simulink model "FOC_Core_OL"  (R2025b)
settings: Solver=FixedStepDiscrete  StartTime=0.0  StopTime=Tstop  FixedStep=8e-05  RelTol=1e-3
undefined symbols (not defined in the file): p
settings Model: Creator=dehc5899  LastModifiedBy=dehc5899
settings SolverCC: AutoInsertRateTranBlk=on
settings DataIOCC: SaveOutput=off  SaveTime=off
settings OptimizationCC: DefaultParameterBehavior=Inlined  EnhancedBackFolding=on  PassReuseOutputArgsAs=Individual arguments  ZeroExternalMemoryAtStartup=off  ZeroInternalMemoryAtStartup=off  OptimizeBlockOrder=speed  DifferentSizesBufferReuse=on  OptimizationCustomize=off  EfficientTunableParamExpr=on
settings DebuggingCC: UnderspecifiedInitializationDetection=Classic  ParameterTunabilityLossMsg=error  BusObjectLabelMismatch=none
settings HardwareCC: ProdBitPerPointer=32.0  ProdBitPerSizeT=32.0  ProdBitPerPtrDiffT=32.0  ProdLargestAtomicInteger=Long  ProdLargestAtomicFloat=Double  ProdWordSize=32.0  ProdHWDeviceType=ARM Compatible->ARM Cortex-M
settings SFSimCC: MATLABDynamicMemAlloc=off
settings RTWCC: SystemTargetFile=ert.tlc  GenCodeOnly=on  GenerateMakefile=off  TemplateMakefile=RTW.MSVCBuild  GenerateReport=on  Description=Create Visual C/C++ Solution File for Embedded Coder
settings CodeAppCC: ForceParamTrailComments=on  IgnoreCustomStorageClasses=off  OperatorAnnotations=on  SimulinkDataObjDesc=on  SFDataObjDesc=on  InsertBlockDesc=on
settings ERTTargetCC: ERTCustomFileTemplate=example_file_process.tlc  TargetLangStandard=C99 (ISO)  GenerateSampleERTMain=on  SupportAbsoluteTime=off  SupportNonFinite=off  SupportComplex=off

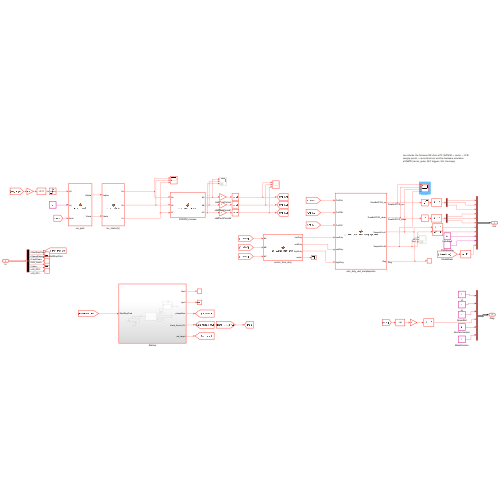
[thumbnail: Simulink's stored preview of the top-level diagram]
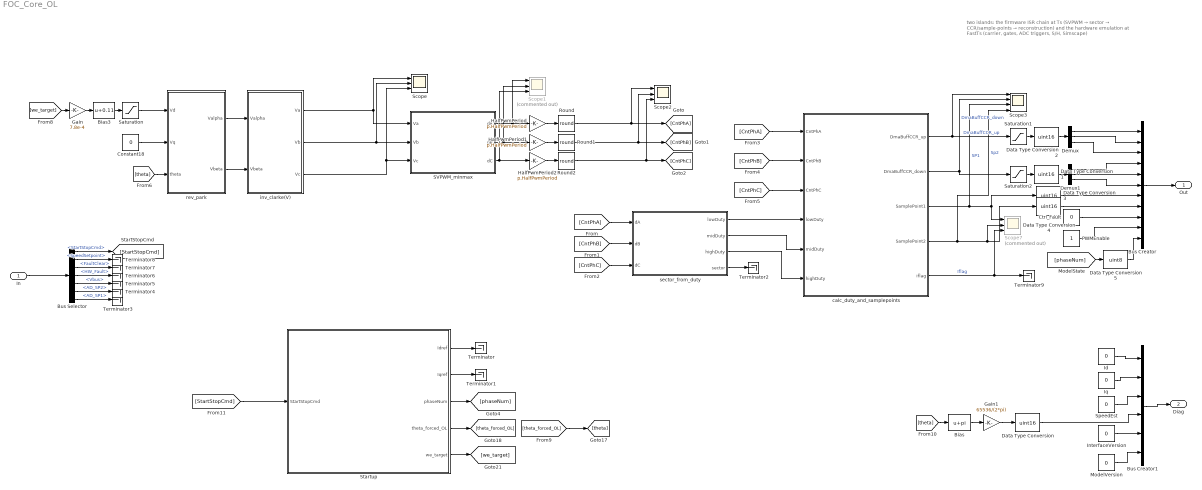
== system FOC_Core_OL ==
  note: two islands: the firmware ISR chain at Ts (SVPWM → sector → CCR/sample-points → reconstruction) and the hardware emulation at FastTs (carrier, gates, ADC triggers, S/H, Simscape)
  In : Inport  OutDataTypeStr=Bus: FOC_Inputs_t
  Bias : Bias  Bias=pi  SaturateOnIntegerOverflow=off
  Bias3 : Bias  Bias=0.11  SaturateOnIntegerOverflow=off
  Bus Creator : BusCreator  Inputs=11  OutDataTypeStr=Bus: FOC_Outputs_t
  Bus Creator1 : BusCreator  Inputs=6  OutDataTypeStr=Bus: FOC_ModelDiag_t
  Bus Selector : BusSelector  OutputSignals=StartStopCmd,SpeedSetpoint,FaultClear,HW_Fault,Vbus,AD_SP2,AD_SP1
  Constant18 : Constant  Value=0
  Ctrl_Fault : Constant  Value=0  OutDataTypeStr=uint16
  Data Type Conversion : DataTypeConversion  OutDataTypeStr=uint16  RndMeth=Floor
  Data Type Conversion{1..4} (4 alike) : DataTypeConversion  OutDataTypeStr=uint16  RndMeth=Nearest
  Data Type Conversion5 : DataTypeConversion  OutDataTypeStr=uint8  RndMeth=Nearest
  Demux : Demux  Outputs=3
  Demux1 : Demux  Outputs=3
  Gain : Gain  Gain=7.8e-4
  Gain1 : Gain  Gain=65536/(2*pi)
  HalfPwmPeriod : Gain  Gain=p.HalfPwmPeriod
  HalfPwmPeriod1 : Gain  Gain=p.HalfPwmPeriod
  HalfPwmPeriod2 : Gain  Gain=p.HalfPwmPeriod
  Id : Constant  Value=0  OutDataTypeStr=int16
  InterfaceVersion : Constant  Value=0  OutDataTypeStr=uint16
  Iq : Constant  Value=0  OutDataTypeStr=int16
  ModelVersion : Constant  Value=0  OutDataTypeStr=uint16
  PWMEnable : Constant  OutDataTypeStr=uint8
  Round : Rounding  Operator=round
  Round1 : Rounding  Operator=round
  Round2 : Rounding  Operator=round
  SVPWM_minmax : MATLAB Function  TreatAsAtomicUnit=on
  Saturation : Saturate  UpperLimit=0.9  LowerLimit=0
  Saturation1 : Saturate  UpperLimit=5120  LowerLimit=0
  Saturation2 : Saturate  UpperLimit=5120  LowerLimit=0
  Scope : Scope  NumInputPorts=3
      settings: ActiveDisplayYMinimum=-1.7670802058532755  ActiveDisplayYMaximum=1.7615871298568744  DataLoggingVariableName=ScopeData24
  Scope1 : Scope  Commented=on  NumInputPorts=3
      settings: ActiveDisplayYMinimum=0.36044361461932012  ActiveDisplayYMaximum=0.40645121419536845  DataLoggingVariableName=ScopeData26
  Scope2 : Scope  NumInputPorts=3
      settings: ActiveDisplayYMinimum=1487.5  ActiveDisplayYMaximum=5312.5  DataLoggingVariableName=ScopeData27
  Scope3 : Scope  NumInputPorts=4
      settings: ActiveDisplayYMinimum=1272.0361133462177  ActiveDisplayYMaximum=3996.5603864724189  DataLoggingVariableName=ScopeData29
  Scope7 : Scope  Commented=on  NumInputPorts=3
      settings: ActiveDisplayYMinimum=669.00000000000011  ActiveDisplayYMaximum=6049  DataLoggingVariableName=ScopeData30
  SpeedEst : Constant  Value=0  OutDataTypeStr=int16
  Startup : Subsystem
  Terminator{,1..9} (10 alike) : Terminator
  calc_duty_and_samplepoints : MATLAB Function  TreatAsAtomicUnit=on
  inv_clarke(V) : MATLAB Function  TreatAsAtomicUnit=on
  rev_park : MATLAB Function  TreatAsAtomicUnit=on
  sector_from_duty : MATLAB Function  TreatAsAtomicUnit=on
  Out : Outport  OutDataTypeStr=Bus: FOC_Outputs_t
  Diag : Outport  Port=2  OutDataTypeStr=Bus: FOC_ModelDiag_t
  wires:
  calc_duty_and_samplepoints/3(SamplePoint1) -> Scope3/3, Data Type Conversion3/1, Scope7/1  "SP1"
  SVPWM_minmax/2(dB) -> Scope1/2, HalfPwmPeriod1/1
  HalfPwmPeriod/1 -> Round/1
  sector_from_duty/3(highDuty) -> calc_duty_and_samplepoints/6(highDuty)
  calc_duty_and_samplepoints/4(SamplePoint2) -> Scope3/4, Data Type Conversion4/1, Scope7/2  "Sp2"
  inv_clarke(V)/2(Vb) -> SVPWM_minmax/2(Vb), Scope/2
  [CntPhC] -> sector_from_duty/3(dC)
  inv_clarke(V)/1(Va) -> Scope/1, SVPWM_minmax/1(Va)
  sector_from_duty/4(sector) -> Terminator2/1
  Round/1 -> [CntPhA], Scope2/1
  HalfPwmPeriod2/1 -> Round2/1
  SVPWM_minmax/3(dC) -> Scope1/3, HalfPwmPeriod2/1
  calc_duty_and_samplepoints/2(DmaBuffCCR_down) -> Saturation2/1, Scope3/2  "DmaBuffCCR_down"
  [CntPhB] -> sector_from_duty/2(dB)
  [CntPhB] -> calc_duty_and_samplepoints/2(CntPhB)
  SVPWM_minmax/1(dA) -> Scope1/1, HalfPwmPeriod/1
  calc_duty_and_samplepoints/1(DmaBuffCCR_up) -> Saturation1/1, Scope3/1  "DmaBuffCCR_up"
  [CntPhA] -> sector_from_duty/1(dA)
  inv_clarke(V)/3(Vc) -> SVPWM_minmax/3(Vc), Scope/3
  Round1/1 -> Scope2/2, [CntPhB]
  sector_from_duty/1(lowDuty) -> calc_duty_and_samplepoints/4(lowDuty)
  [CntPhC] -> calc_duty_and_samplepoints/3(CntPhC)
  sector_from_duty/2(midDuty) -> calc_duty_and_samplepoints/5(midDuty)
  [CntPhA] -> calc_duty_and_samplepoints/1(CntPhA)
  HalfPwmPeriod1/1 -> Round1/1
  Round2/1 -> Scope2/3, [CntPhC]
  calc_duty_and_samplepoints/5(iflag) -> Terminator9/1, Scope7/3  "Iflag"
  [we_target] -> Gain/1
  Startup/3(phaseNum) -> [phaseNum]
  Constant18/1 -> rev_park/2(Vq)
  Startup/5(we_target) -> [we_target]
  Gain/1 -> Bias3/1
  [theta_forced_OL] -> [theta]
  Saturation/1 -> rev_park/1(Vd)
  rev_park/1(Valpha) -> inv_clarke(V)/1(Valpha)
  Startup/4(theta_forced_OL) -> [theta_forced_OL]
  rev_park/2(Vbeta) -> inv_clarke(V)/2(Vbeta)
  Startup/2(Iqref) -> Terminator1/1
  [theta] -> rev_park/3(theta)
  Startup/1(Idref) -> Terminator/1
  Bias3/1 -> Saturation/1
  In/1 -> Bus Selector/1
  Bus Selector/7 -> Terminator3/1  "<AD_SP1>"
  Bus Selector/6 -> Terminator4/1  "<AD_SP2>"
  Bus Selector/5 -> Terminator5/1  "<Vbus>"
  Bus Selector/4 -> Terminator6/1  "<HW_Fault>"
  Bus Selector/3 -> Terminator7/1  "<FaultClear>"
  Bus Selector/2 -> Terminator8/1  "<SpeedSetpoint>"
  Bus Selector/1 -> [StartStopCmd]  "<StartStopCmd>"
  Demux/1 -> Bus Creator/1
  Demux/2 -> Bus Creator/2
  Demux/3 -> Bus Creator/3
  Demux1/1 -> Bus Creator/4
  Demux1/2 -> Bus Creator/5
  Demux1/3 -> Bus Creator/6
  Ctrl_Fault/1 -> Bus Creator/9
  PWMEnable/1 -> Bus Creator/10
  [phaseNum] -> Data Type Conversion5/1
  Bus Creator/1 -> Out/1
  Saturation1/1 -> Data Type Conversion2/1
  Saturation2/1 -> Data Type Conversion1/1
  Id/1 -> Bus Creator1/1
  Iq/1 -> Bus Creator1/2
  Bus Creator1/1 -> Diag/1
  InterfaceVersion/1 -> Bus Creator1/5
  ModelVersion/1 -> Bus Creator1/6
  [theta] -> Bias/1
  Bias/1 -> Gain1/1
  Gain1/1 -> Data Type Conversion/1
  Data Type Conversion/1 -> Bus Creator1/4
  [StartStopCmd] -> Startup/1(StartStopCmd)
  SpeedEst/1 -> Bus Creator1/3
  Data Type Conversion1/1 -> Demux1/1
  Data Type Conversion2/1 -> Demux/1
  Data Type Conversion3/1 -> Bus Creator/7
  Data Type Conversion4/1 -> Bus Creator/8
  Data Type Conversion5/1 -> Bus Creator/11

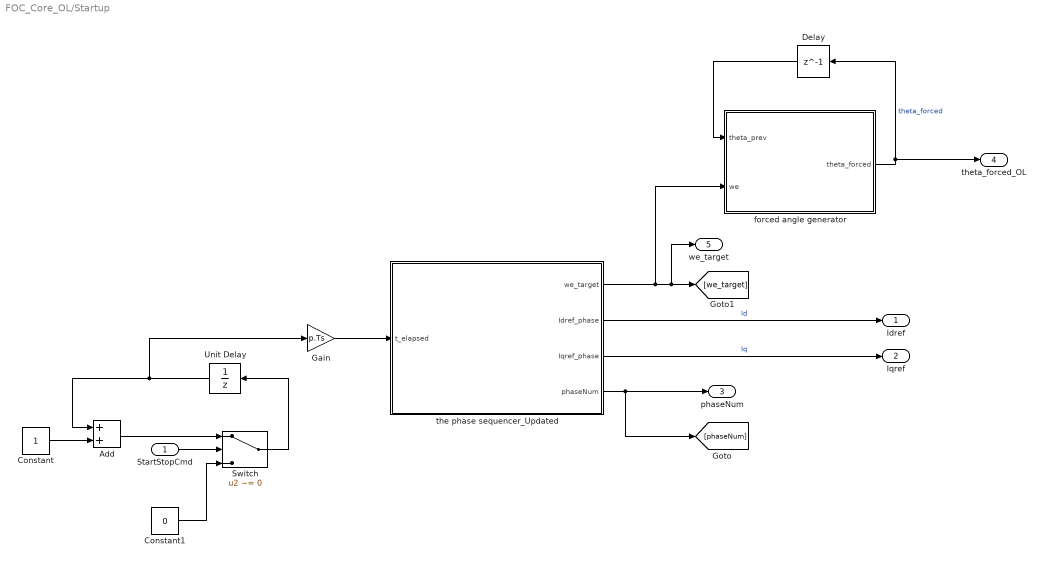
== system FOC_Core_OL/Startup ==
  StartStopCmd : Inport
  Add : Sum
  Constant : Constant  OutDataTypeStr=uint32
  Constant1 : Constant  Value=0  OutDataTypeStr=uint32
  Delay : Delay  DelayLength=1  SampleTime=p.Ts
  Gain : Gain  Gain=p.Ts  ParamDataTypeStr=double  OutDataTypeStr=double
  Switch : Switch  Criteria=u2 ~= 0  SaturateOnIntegerOverflow=off  InputSameDT=off
  Unit Delay : UnitDelay  SampleTime=-1  HasFrameUpgradeWarning=on
  forced angle generator : MATLAB Function  TreatAsAtomicUnit=on
  the phase sequencer_Updated : MATLAB Function  TreatAsAtomicUnit=on
  Idref : Outport
  Iqref : Outport  Port=2
  phaseNum : Outport  Port=3  OutDataTypeStr=double
  theta_forced_OL : Outport  Port=4
  we_target : Outport  Port=5
  wires:
  the phase sequencer_Updated/1(we_target) -> [we_target], we_target/1, forced angle generator/2(we)
  the phase sequencer_Updated/2(Idref_phase) -> Idref/1  "Id"
  the phase sequencer_Updated/3(Iqref_phase) -> Iqref/1  "Iq"
  Delay/1 -> forced angle generator/1(theta_prev)
  forced angle generator/1(theta_forced) -> theta_forced_OL/1, Delay/1  "theta_forced"
  the phase sequencer_Updated/4(phaseNum) -> [phaseNum], phaseNum/1
  Constant/1 -> Add/2
  Unit Delay/1 -> Add/1, Gain/1
  Gain/1 -> the phase sequencer_Updated/1(t_elapsed)
  Add/1 -> Switch/1
  StartStopCmd/1 -> Switch/2
  Constant1/1 -> Switch/3
  Switch/1 -> Unit Delay/1

== matlab function FOC_Core_OL/SVPWM_minmax ==
  data: Va input; dA output; Vb input; Vc input; dB output; dC output
function [dA, dB, dC] = ss_svpwm_minmax(Va, Vb, Vc)
%SS_SVPWM_MINMAX Carrier-based SVPWM via min-max common-mode injection.
%
% Standard trick to get space-vector-equivalent modulation without ever
% computing a vector angle or sector: subtract the average of the largest
% and smallest of the three instantaneous reference voltages from all
% three. That "third-harmonic-like" zero-sequence term cancels line-to-
% line (so it doesn't affect the actual motor voltages) but centers the
% three duty cycles inside the 0..1 carrier range, extending the linear
% modulation range from m=1 (plain sine-triangle) to m=2/sqrt(3)~=1.1547
% (six-step limit) - the same range single-shunt SVPWM assumes.
%
% This is the same formula used inline in
% test_single_shunt_reconstruction.m (and export_for_simulink.m); pulled
% out here so it can be dropped into a Simulink MATLAB Function block and
% reused instead of duplicated.
%
% Va, Vb, Vc : per-unit reference phase voltages, nominally in [-1, 1]
%              (e.g. Va = m*cos(theta_e), 120 deg apart), where m is the
%              modulation index.
%
% dA, dB, dC : duty cycle in [0, 1], ready for the next stage (converting
%              to timer counter/CCR values, i.e. CntPhX = round(dX *
%              Half_PWMPeriod) - NOT done here on purpose, kept as a
%              separate step).

v0 = -(max([Va, Vb, Vc]) + min([Va, Vb, Vc])) / 2;

dA = 0.5 + 0.5 * (Va + v0);
dB = 0.5 + 0.5 * (Vb + v0);
dC = 0.5 + 0.5 * (Vc + v0);

end

== matlab function FOC_Core_OL/calc_duty_and_samplepoints ==
  data: CntPhA input; DmaBuffCCR_up output size=[1 3]; CntPhB input; CntPhC input; lowDuty input; midDuty input; highDuty input; DmaBuffCCR_down output size=[1 3]; SamplePoint1 output; SamplePoint2 output; iflag output; p parameter
function [DmaBuffCCR_up, DmaBuffCCR_down, SamplePoint1, SamplePoint2, iflag] = ...
    ss_calc_duty_and_samplepoints(CntPhA, CntPhB, CntPhC, lowDuty, midDuty, highDuty, p)
%SS_CALC_DUTY_AND_SAMPLEPOINTS MATLAB port of R1_CalcDutyCycles()
% (Src/r1_ps_pwm_curr_fdbk.c, ~lines 1097-1282).
%
% Every PWM period, single-shunt sensing needs two ADC injected
% conversions of the DC-link shunt current, timed to fall inside the two
% "two-phases-on" sub-intervals either side of the mid-duty phase's
% switching edges. Those windows only exist, and are only wide enough to
% trigger + finish a conversion (>= p.TMin ticks), when the three duty
% cycles are far enough apart. Close to a sector boundary (two duties
% nearly equal) the natural window collapses, so this function:
%
%   1) checks the two natural gaps (high-mid, mid-low) against TMin;
%   2) if a gap is too small but can still be opened by shifting the
%      shorter leg's compare value by a few ticks, does so via aShiftval
%      (kept symmetric: +shift in the first half of the center-aligned
%      PWM period, -shift in the second half, so the AVERAGE duty over
%      the full period - and thus the commanded voltage - is unchanged);
%   3) if even that isn't possible (duty pinned near 0% or 100%), marks
%      that phase as unavailable this period (iflag bit cleared) and
%      falls back to one fixed sampling point at mid-period;
%   4) returns iflag (IA_OK/IB_OK/IC_OK bits) telling
%      ss_get_phase_currents() which phase current(s) can be trusted from
%      this period's two ADC samples, and which must fall back to an
%      estimate instead.
%
% Inputs are all timer ticks (see ss_params, matches p.HalfPwmPeriod).
% CntPhA/B/C : commanded compare values (0..p.HalfPwmPeriod)
% lowDuty/midDuty/highDuty : 0-based phase index (0=A,1=B,2=C), from
%                            ss_sector_from_duty
%
% Outputs:
% DmaBuffCCR_up/down : shifted CCR values for the up-count / down-count
%                      half of the period (mirrors DmaBuffCCR[0:2] and
%                      DmaBuffCCR[4:6])
% SamplePoint1/2     : ADC trigger points in timer ticks (TIM1_CH5/CH6)
% iflag              : uint8 bitmask, bit0=IA_OK bit1=IB_OK bit2=IC_OK

IA_OK = uint8(1); IB_OK = uint8(2); IC_OK = uint8(4);
ALFLAG = [IA_OK IB_OK IC_OK];

aCCRval = [CntPhA, CntPhB, CntPhC];
maxVal = highDuty + 1;   % to 1-based MATLAB index
midIdx = midDuty  + 1;
minVal = lowDuty  + 1;

iflag = uint8(0);
aShiftval = [0 0 0];

submax_mid          = aCCRval(maxVal) - aCCRval(midIdx);
submax_mid_deltmin   = submax_mid - p.TMin;
submid_min           = aCCRval(midIdx) - aCCRval(minVal);
submid_min_deltmin   = submid_min - p.TMin;
max_bad_flag = false;
min_bad_flag = false;

if submax_mid_deltmin > 0
    iflag = bitor(iflag, ALFLAG(maxVal));
else
    if (1 - submax_mid_deltmin + aCCRval(maxVal) + p.hTADConv) > p.HalfPwmPeriod
        max_bad_flag = true;            % no room to open a window even after shifting
    else
        iflag = bitor(iflag, ALFLAG(maxVal));
        aShiftval(maxVal) = 1 - submax_mid_deltmin;
    end
end

if submid_min_deltmin > 0
    iflag = bitor(iflag, ALFLAG(minVal));
else
    if (submid_min_deltmin - 1 + aCCRval(minVal)) < 0
        min_bad_flag = true;
    else
        iflag = bitor(iflag, ALFLAG(minVal));
        aShiftval(minVal) = submid_min_deltmin - 1;
    end
end

if (~max_bad_flag) && (~min_bad_flag)
    SamplePoint1 = aCCRval(midIdx) - p.TSample;
    SamplePoint2 = aCCRval(midIdx) + p.TMin - p.TSample;
elseif max_bad_flag && min_bad_flag
    SamplePoint1 = p.HalfPwmPeriod / 2;
    SamplePoint2 = SamplePoint1 + p.TSample + p.hTADConv;
elseif max_bad_flag
    SamplePoint1 = aCCRval(midIdx) - p.TSample;
    SamplePoint2 = aCCRval(midIdx) + p.hTADConv;
else
    SamplePoint2 = aCCRval(midIdx) + p.TMin - p.TSample;
    SamplePoint1 = aCCRval(midIdx);
end


if (SamplePoint2 - SamplePoint1) < p.hTADConv
    iflag = bitand(iflag, ALFLAG(maxVal));
    iflag = bitand(iflag, bitcmp(ALFLAG(minVal)));
    SamplePoint1 = p.HalfPwmPeriod / 2;
    SamplePoint2 = SamplePoint1 + p.TSample + p.hTADConv;
end

if (SamplePoint2 >= p.HalfPwmPeriod) || (SamplePoint2 <= 0)
    iflag = bitand(iflag, ALFLAG(maxVal));
    SamplePoint2 = aCCRval(midIdx) + p.hTADConv;
end
if (SamplePoint1 >= p.HalfPwmPeriod) || (SamplePoint1 <= 0)
    iflag = bitand(iflag, bitcmp(ALFLAG(minVal)));
    SamplePoint1 = aCCRval(midIdx);
end

DmaBuffCCR_up   = [CntPhA, CntPhB, CntPhC] + aShiftval;   % up-count half   (DmaBuffCCR[0:2])
DmaBuffCCR_down = [CntPhA, CntPhB, CntPhC] - aShiftval;   % down-count half (DmaBuffCCR[4:6])

end

== matlab function FOC_Core_OL/sector_from_duty ==
  data: dA input; lowDuty output; dB input; dC input; midDuty output; highDuty output; sector output
function [lowDuty, midDuty, highDuty, sector] = ss_sector_from_duty(dA, dB, dC)
%SS_SECTOR_FROM_DUTY Single-shunt "sector" (1-6) from the ranking of the
% three phase duty cycles, plus the low/mid/high phase-index table used by
% the firmware's SingleShuntTopology branch.
%
% Source: Src/pwm_curr_fdbk.c, PWMC_SetPhaseVoltage() (~lines 190-320).
% For SingleShuntTopology==true, ST hard-codes lowDuty/midDuty/highDuty
% per sector instead of sorting the duty values at runtime:
%
%   SECTOR_1: low=C(2) mid=B(1) high=A(0)
%   SECTOR_2: low=C(2) mid=A(0) high=B(1)
%   SECTOR_3: low=A(0) mid=C(2) high=B(1)
%   SECTOR_4: low=A(0) mid=B(1) high=C(2)
%   SECTOR_5: low=B(1) mid=A(0) high=C(2)
%   SECTOR_6: low=B(1) mid=C(2) high=A(0)
%
% Those 6 fixed tables are simply the 6 possible strict orderings of
% (A,B,C) duty - which is exactly what single-shunt sampling cares about,
% since it is the ORDER the three legs switch in (not the SVM angle
% itself) that determines which phase current flows through the shunt
% during each sub-interval. Ranking the actual duty values here is
% therefore equivalent to, but independent of, ST's fixed-point angle
% (wX/wY/wZ) sector computation - it removes any risk of an angle-
% convention mismatch while producing identical low/mid/high results for
% any physically valid duty pattern.
%
% dA, dB, dC : commanded ON-time duty of phase A/B/C, any consistent unit
%              (ticks or 0..1), this period.
%
% Returns 0-based phase indices (0=A, 1=B, 2=C) for lowDuty/midDuty/highDuty,
% matching pHandle->lowDuty/midDuty/highDuty in the C driver.

d = [dA, dB, dC];
[~, order] = sort(d);              % order(1) = index(1-based) of smallest duty
low  = order(1) - 1;
mid  = order(2) - 1;
high = order(3) - 1;

table = [ 2 1 0;   % SECTOR_1
          2 0 1;   % SECTOR_2
          0 2 1;   % SECTOR_3
          0 1 2;   % SECTOR_4
          1 0 2;   % SECTOR_5
          1 2 0 ]; % SECTOR_6

sector = 1;                       % default, same as the old else branch
for k = 1:6
    if all(table(k,:) == [low mid high])
        sector = k;
        break;
    end
end
lowDuty = low;
midDuty = mid;
highDuty = high;
end

== matlab function FOC_Core_OL/Startup/forced angle generator ==
  data: theta_prev input; theta_forced output; we input; p parameter
function theta_forced  = ss_theta_step(theta_prev, we, p)
%SS_THETA_STEP Open-loop electrical angle generator (bench-test stand-in
% for the sensorless STO-PLL observer, sto_pll_speed_pos_fdbk.c, which
% isn't wired into this testbed). Integrates a commanded electrical speed
% `we` [rad/s] once per PWM period and wraps to (-pi, pi], exactly the
% "forced angle" mode used to bring up a current loop before closing the
% speed/position loop on a real drive.
%
% theta_prev : previous period's angle (radians) - feed from a Unit Delay
%              (Z^-1), initial condition 0, same as IaEst/IbEst/IcEst
% we         : commanded electrical speed, rad/s (2*pi*fe)
% Ts         : p.Ts (must match the model's execution rate)

theta_forced  = theta_prev + we * p.Ts;
theta_forced  = mod(theta_forced  + pi, 2*pi) - pi;

end

== matlab function FOC_Core_OL/Startup/the phase sequencer_Updated ==
  data: t_elapsed input; we_target output; Idref_phase output; Iqref_phase output; phaseNum output; p parameter
function [we_target, Idref_phase, Iqref_phase, phaseNum] = ss_startup_sequencer(t_elapsed, p)
%SS_STARTUP_SEQUENCER Smooth-transition startup sequencer for loaded motor
%
% Phase Breakdown:
%   Phase 1 (Align)       : 0.000 - 0.200 s | Holds 0 RPM | Id = 10A, Iq = 0A
%   Phase 1.5 (Transition): 0.200 - 0.220 s | Holds 0 RPM | Id ramps 10A->0A, Iq ramps 0A->10A
%   Phase 2 (Ramp/Acc)    : 0.220 - 0.620 s | Ramps to 2500 RPM | Iq tapers 10A->8A
%   Phase 3               : 0.620 - 0.621 s | Ramps to 2510 RPM | Iq = 8A
%   Phase 4               : 0.621 - 0.622 s | Ramps to 2520 RPM | Iq = 8A
%   Phase 5               : 0.622 - 0.623 s | Ramps to 2530 RPM | Iq = 8A
%   Phase 6               : > 0.623 s       | Ready for closed-loop handover

rpm2we = (2*pi/60) * p.MotorPolePairs;
we_bkpts = p.Startup_RPM * rpm2we;
t_bkpts  = [0, p.Startup_T];

% 1. Command open-loop target electrical speed (we_target)
t_clamped = min(t_elapsed, p.Startup_T(end));
we_target = interp1(t_bkpts, we_bkpts, t_clamped, 'linear');

% 2. Current Reference and Phase State Machine
T_align = p.Startup_T(1); % End of pure align
T_blend = p.Startup_T(2); % End of Id -> Iq blend duration

if t_elapsed <= T_align
    % --- PHASE 1: Pure Alignment (DC Lock) ---
    phaseNum = 1;
    Idref_phase = p.Startup_Id_A;
    Iqref_phase = 0;

elseif t_elapsed <= T_blend
    % --- PHASE 1.5: Smooth Vector Blend (Soft-Transfer at Standstill) ---
    phaseNum = 1.5;
    % Normalized alpha factor going from 0 -> 1 over the blend time
    alpha = (t_elapsed - T_align) / (T_blend - T_align);
    
    % Smooth cross-fade between Id and Iq to avoid current step spikes
    Idref_phase = (1 - alpha) * p.Startup_Id_A;
    Iqref_phase = alpha * p.Startup_Iq_Breakaway_A;

elseif t_elapsed <= p.Startup_T(3)
    % --- PHASE 2: Main Acceleration Ramp ---
    phaseNum = 2;
    Idref_phase = 0;
    
    % Taper Iq down from Breakaway Torque (10A) to Running Startup Torque (4A)
    % as speed increases and static friction drops to dynamic friction
    T_ramp_start = T_blend;
    T_ramp_end   = p.Startup_T(3);
    beta = (t_elapsed - T_ramp_start) / (T_ramp_end - T_ramp_start);
    
    Iqref_phase = (1 - beta) * p.Startup_Iq_Breakaway_A + beta * p.Startup_Iq_A;

elseif t_elapsed <= p.Startup_T(4)
    % --- PHASE 3 ---
    phaseNum = 3;
    Idref_phase = 0;
    Iqref_phase = p.Startup_Iq_A;

elseif t_elapsed <= p.Startup_T(5)
    % --- PHASE 4 ---
    phaseNum = 4;
    Idref_phase = 0;
    Iqref_phase = p.Startup_Iq_A;

elseif t_elapsed <= p.Startup_T(6)
    % --- PHASE 5 ---
    phaseNum = 5;
    Idref_phase = 0;
    Iqref_phase = p.Startup_Iq_A;

else
    % --- PHASE 6: Observer Handoff Ready ---
    phaseNum = 6;
    Idref_phase = 0;
    Iqref_phase = p.Startup_Iq_A; % Holds constant; superseded by Speed Loop Iqref once closed
end

end

== matlab function FOC_Core_OL/inv_clarke(V) ==
  data: Valpha input; Va output; Vbeta input; Vb output; Vc output
function [Va, Vb, Vc] = ss_inv_clarke(Valpha, Vbeta)
%SS_INV_CLARKE Inverse Clarke transform - NOT a firmware port (the real
% MCSDK has no such function: PWMC_SetPhaseVoltage() computes SVM duty
% directly from alpha-beta via the fixed-point wX/wY/wZ method, never
% forming Va/Vb/Vc explicitly). This is the bridge WE need because
% ss_svpwm_minmax.m (the SVPWM stage already validated in this build)
% works in the three-phase domain rather than being a byte-for-byte port
% of that alpha-beta-native method (see ss_sector_from_duty.m header).
%
% Derived as the exact algebraic inverse of ss_clarke.m's specific sign
% convention (Ibeta = -(Ia+2*Ib)/sqrt(3), i.e. flipped vs. the "textbook"
% Clarke transform) - NOT copied from a generic inverse-Clarke formula,
% to guarantee round-tripping through ss_clarke.m -> ss_park.m ->
% ss_rev_park.m -> here reproduces the original three phases exactly.
% Verified: ss_inv_clarke(ss_clarke(Ia,Ib)) == [Ia, Ib, Ic] for any Ia,Ib.
%
% Valpha, Vbeta : ss_rev_park.m output (per-unit stationary-frame voltage)
% Va, Vb, Vc    : per-unit three-phase reference voltage, same scale/sign
%                 convention as the Va/Vb/Vc already feeding
%                 ss_svpwm_minmax.m

Va = Valpha;
Vb = -Valpha/2 - (sqrt(3)/2) * Vbeta;
Vc = -Valpha/2 + (sqrt(3)/2) * Vbeta;

end

== matlab function FOC_Core_OL/rev_park ==
  data: Vd input; Valpha output; Vq input; theta input; Vbeta output
function [Valpha, Vbeta] = ss_rev_park(Vd, Vq, theta)
%SS_REV_PARK MATLAB port of MCM_Rev_Park() (Src/mc_math.c, ~lines
% 258-297): Valpha = Vq*cos(theta) + Vd*sin(theta)
%           Vbeta  = -Vq*sin(theta) + Vd*cos(theta)
%
% Exact inverse of ss_park.m under the same convention (verified when
% Park was written: Rev_Park(Park(Ialpha,Ibeta,theta),theta) = Ialpha,
% Ibeta for any theta).
%
% Vd, Vq : synchronous-frame voltage commands (PI controller outputs,
%          already converted to per-unit via p.VoltageFullScale)
% theta  : rotor electrical angle, radians (same theta fed to ss_park.m)

c = cos(theta);
s = sin(theta);

Valpha = Vq * c + Vd * s;
Vbeta  = -Vq * s + Vd * c;

end
